simulink subsystem "LQR_Gain_Scheduler"  (R2026a)
settings: Solver=VariableStepAuto
settings Model: Creator=asing  LastModifiedBy=asing

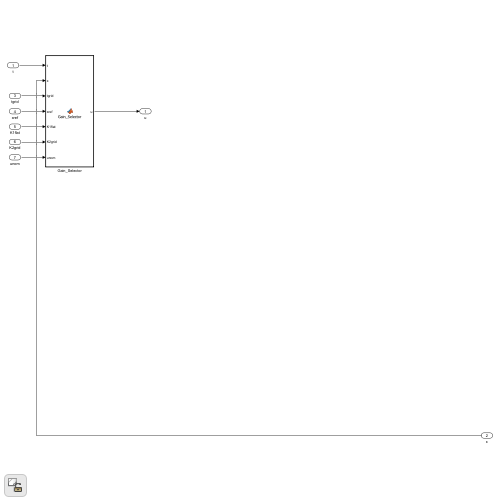
[thumbnail: Simulink's stored preview of the top-level diagram]
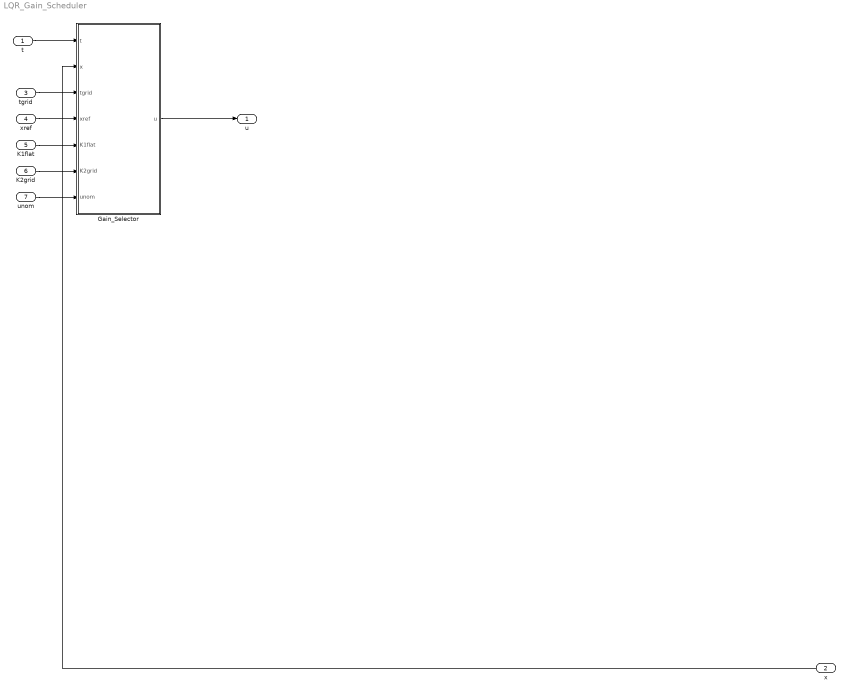
== system LQR_Gain_Scheduler ==
  t : Inport
  x : Inport  Port=2
  tgrid : Inport  Port=3
  xref : Inport  Port=4
  K1flat : Inport  Port=5
  K2grid : Inport  Port=6
  unom : Inport  Port=7
  Gain_Selector : MATLAB Function  TreatAsAtomicUnit=on
  u : Outport
  wires:
  unom/1 -> Gain_Selector/7(unom)
  K2grid/1 -> Gain_Selector/6(K2grid)
  K1flat/1 -> Gain_Selector/5(K1flat)
  tgrid/1 -> Gain_Selector/3(tgrid)
  t/1 -> Gain_Selector/1(t)
  xref/1 -> Gain_Selector/4(xref)
  x/1 -> Gain_Selector/2(x)
  Gain_Selector/1(u) -> u/1

== matlab function LQR_Gain_Scheduler/Gain_Selector ==
  data: t input; u output; x input; tgrid input; xref input; K1flat input; K2grid input; unom input
function u = Gain_Selector(t, x, tgrid, xref, K1flat, K2grid, unom)
%#codegen
% Fixed-size output: u is always 4x1

u = zeros(4,1);

x = x(:);              % should be 13x1 for 6DOF
N = length(tgrid);

% --- Clamp time and compute interval index ---
if t <= tgrid(1)
    idx = 1;
    w = 0.0;
elseif t >= tgrid(end)
    idx = N-1;
    w = 1.0;
else
    idx = 1;
    for k = 1:(N-1)
        if tgrid(k) <= t && t < tgrid(k+1)
            idx = k;
            break;
        end
    end
    t1 = tgrid(idx);
    t2 = tgrid(idx+1);
    w  = (t - t1) / (t2 - t1);
end

% --- Interpolate reference state (13x1) ---
xref_t = (1-w)*xref(idx,:)' + w*xref(idx+1,:)';

% --- Interpolate K1flat then reshape to 4x13 ---
Kflat = (1-w)*K1flat(idx,:) + w*K1flat(idx+1,:);
K1 = reshape(Kflat, 13, 4)';   % 4x13   (requires K1flat is N×52)

% --- Interpolate K2 (4x1) ---
K2 = (1-w)*K2grid(idx,:)' + w*K2grid(idx+1,:)';

% --- Interpolate nominal control (4x1) ---
u_nom = (1-w)*unom(idx,:)' + w*unom(idx+1,:)';

q     = x(10:13);
qref  = xref_t(10:13);

if dot(q,qref) < 0
    q = -q;
end

x_used = x;
x_used(10:13) = q;

dx = x_used - xref_t;


% --- Control law ---
%dx = (x - xref_t);          % 13x1
u  =u_nom+(-K1*dx)-K2;  
%fix

end
